simulink model "control_tsc_planta"  (R2024a)
settings: Solver=ode15s  StartTime=0.0  StopTime=tm_final  MaxStep=tm_h  RelTol=1e-9  AbsTol=1e-11
model workspace (MAT data in the model file):
  tm_C1 = 1.87501784269e-05
  tm_C2 = 3.75003568539e-05
  tm_Cp = 2.89288467158e-06
  tm_L1 = 0.26018031666
  tm_L2 = 0.13009015833
  tm_PNominal_W = 1000
  tm_R1 = 1.15690788571
  tm_R2 = 0.578453942857
  tm_Rb1 = 84640
  tm_Rb2 = 42320
  tm_Rp = 2.20064
  tm_Urms = 230
  tm_a1 = 1
  tm_a2 = 0.03
  tm_a3 = 0.03
  tm_carga = [0 0.0001 0.0002 0.0003 0.0004 0.0005 0.0006 0.0007 0.0008 0.0009 0.001 0.0011 ... (16020 elements, 8010x2)]
  tm_final = 0.8
  tm_h = 2.5e-05
  tm_lambda = 229.793279031
  tm_modes = [0  0  0; 0.0351508783586  0  0; 0.0351508783586  1  0; 0.248585882825  1  0; 0.248585882825  0  0; 0.255150878358  0  0; 0.255150878358  0  1; 0.3300515321  0  1; 0.3300515321  1  1; 0.450321519106  1  1; 0.450321519106  0  1; 0.530051552275  0  1; 0.530051552275  1  1; 0.531472138746  1  1; 0.531472138746  1  0; 0.640194068677  1  0; 0.640194068677  0  0; 0.650055060945  0  0; 0.650055060945  0  1; 0.8  0  1]
  tm_omega = 314.159265359
  tm_outputtimes = [0 0.0001 0.0002 0.0003 0.0004 0.0005 0.0006 0.0007 0.0008 0.0009 0.001 0.0011 ... (8014 elements, 8014x1)]
  tm_vC10 = 0
  tm_vC20 = 0
  tm_vCp0 = 344.473571203
(part 1 of 2)
Description:
  | Auditoria de planta: RC fijo y dos LC con R serie y descarga Rb. Integra estados fisicos usando el cronograma ON/OFF aplicado externamente. No contiene el supervisor GA ni modelos de semiconductor. VC es continuo. Una desconexion presupone corriente cero y su residuo se audita. Fuente 230 V RMS; escala de potencia nominal 1000 W. Coeficientes de tension [1 0.03 0.03].
settings Model: Creator=paco  LastModifiedBy=paco
settings DataIOCC: SaveOutput=off  SignalLogging=off  SaveTime=off  OutputOption=SpecifiedOutputTimes  OutputTimes=tm_outputtimes

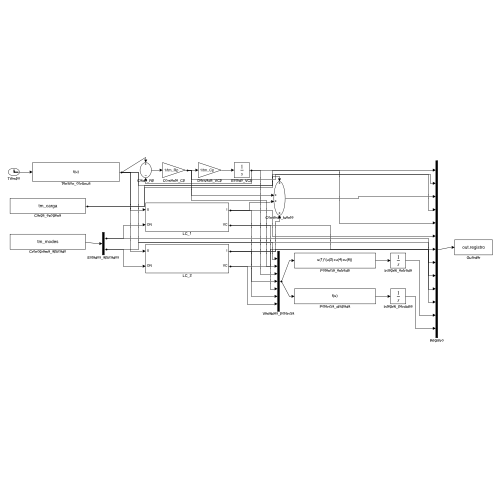
[thumbnail: Simulink's stored preview of the top-level diagram]
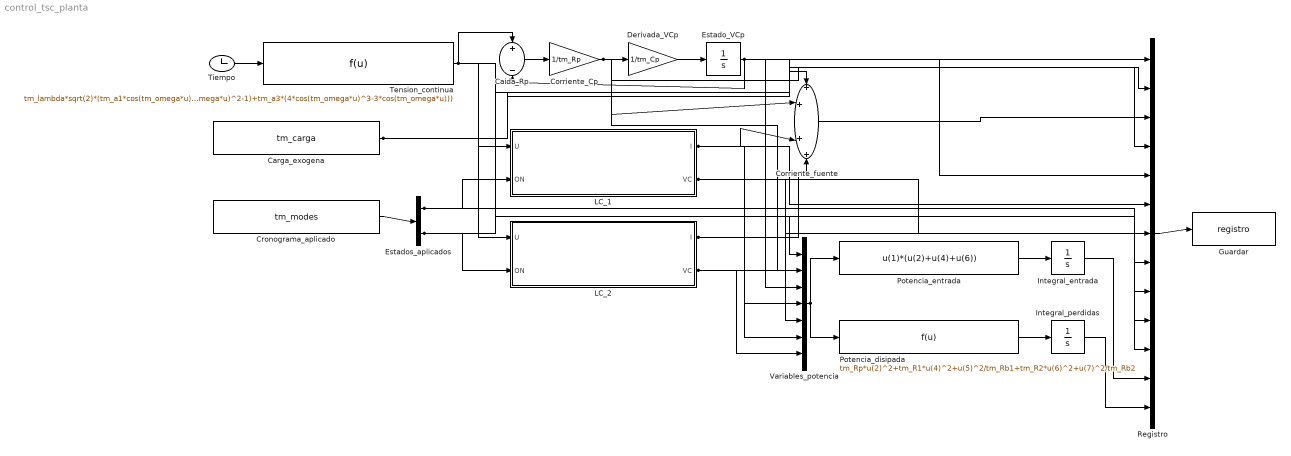
== system control_tsc_planta ==
  Caida_Rp : Sum  Inputs=+-
  Carga_exogena : FromWorkspace  VariableName=tm_carga  OutputAfterFinalValue=Holding final value
  Corriente_Cp : Gain  Gain=1/tm_Rp
  Corriente_fuente : Sum  Inputs=++++
  Cronograma_aplicado : FromWorkspace  VariableName=tm_modes  OutputAfterFinalValue=Holding final value
  Derivada_VCp : Gain  Gain=1/tm_Cp
  Estado_VCp : Integrator  InitialCondition=tm_vCp0
  Estados_aplicados : Demux  Outputs=2
  Guardar : ToWorkspace  VariableName=registro  SaveFormat=Timeseries  SampleTime=-1
  Integral_entrada : Integrator
  Integral_perdidas : Integrator
  LC_1 : Subsystem
  LC_2 : Subsystem
  Potencia_disipada : Fcn  Expr=tm_Rp*u(2)^2+tm_R1*u(4)^2+u(5)^2/tm_Rb1+tm_R2*u(6)^2+u(7)^2/tm_Rb2
  Potencia_entrada : Fcn  Expr=u(1)*(u(2)+u(4)+u(6))
  Registro : Mux  Inputs=13
  Tension_continua : Fcn  Expr=tm_lambda*sqrt(2)*(tm_a1*cos(tm_omega*u)+tm_a2*(2*cos(tm_omega*u)^2-1)+tm_a3*(4*cos(tm_omega*u)^3-3*cos(tm_omega*u)))
  Tiempo : Clock
  Variables_potencia : Mux  Inputs=7
  wires:
  Tiempo/1 -> Tension_continua/1
  Tension_continua/1 -> Caida_Rp/1, LC_1/1(U), LC_2/1(U), Variables_potencia/1, Registro/1
  Estado_VCp/1 -> Caida_Rp/2, Variables_potencia/3, Registro/5
  Caida_Rp/1 -> Corriente_Cp/1
  Corriente_Cp/1 -> Derivada_VCp/1, Corriente_fuente/2, Variables_potencia/2, Registro/4
  Derivada_VCp/1 -> Estado_VCp/1
  Cronograma_aplicado/1 -> Estados_aplicados/1
  Carga_exogena/1 -> Corriente_fuente/1, Registro/2
  Estados_aplicados/1 -> LC_1/2(ON), Registro/10
  LC_1/1(I) -> Corriente_fuente/3, Variables_potencia/4, Registro/6
  Estados_aplicados/2 -> LC_2/2(ON), Registro/11
  LC_2/1(I) -> Corriente_fuente/4, Variables_potencia/6, Registro/8
  LC_1/2(VC) -> Variables_potencia/5, Registro/7
  LC_2/2(VC) -> Variables_potencia/7, Registro/9
  Variables_potencia/1 -> Potencia_entrada/1, Potencia_disipada/1
  Potencia_entrada/1 -> Integral_entrada/1
  Potencia_disipada/1 -> Integral_perdidas/1
  Corriente_fuente/1 -> Registro/3
  Integral_entrada/1 -> Registro/12
  Integral_perdidas/1 -> Registro/13
  Registro/1 -> Guardar/1
